simulink model "Powertrain_Comparison"  (R2024b)
settings: Solver=FixedStepDiscrete  StartTime=0.0  StopTime=3600  FixedStep=1  RelTol=1e-3
InitFcn:
  | try; sc=find_system(bdroot,'LookUnderMasks','all','FollowLinks','on','BlockType','Scope'); for k=1:numel(sc); c=get_param(sc{k},'ScopeConfiguration'); try; c.AxesScaling='Auto'; catch; end; try; nd=prod(c.LayoutDimensions); catch; nd=1; end; for d=1:nd; try; c.ActiveDisplay=d; catch; end; try; c.ShowLegend=true; catch; end; end; end; catch; end
(part 4 of 4)

== system Powertrain_Comparison/Electric powertrain/Battery storage/Battery management/Stored_energy_inventory ==
  note: Stored energy inventory
  note: OUTPUTS AND MONITORING
  SOC_fraction : Inport  PortDimensions=1
  OCV_segment_1 : Fcn  Expr=ocv_cell_V(1)*(((((u(1)-ocv_soc(1))+abs(u(1)-ocv_soc(1)))/2)+(ocv_soc(2)-ocv_soc(1))-abs((((u(1)-ocv_soc(1))+abs(u(1)-ocv_soc(1)))/2)-(ocv_soc(2)-ocv_soc(1))))/2)+0.5*(ocv_cell_V(2)-ocv_cell_V(1))/(ocv_soc(2)-ocv_soc(1))*(((((u(1)-ocv_soc(1))+abs(u(1)-ocv_soc(1)))/2)+(ocv_soc(2)-ocv_soc(1))-abs((((u(1)-ocv_soc(1))+abs(u(1)-ocv_soc(1)))/2)-(ocv_soc(2)-ocv_soc(1))))/2)^2
  OCV_segment_10 : Fcn  Expr=ocv_cell_V(10)*(((((u(1)-ocv_soc(10))+abs(u(1)-ocv_soc(10)))/2)+(ocv_soc(11)-ocv_soc(10))-abs((((u(1)-ocv_soc(10))+abs(u(1)-ocv_soc(10)))/2)-(ocv_soc(11)-ocv_soc(10))))/2)+0.5*(ocv_cell_V(11)-ocv_cell_V(10))/(ocv_soc(11)-ocv_soc(10))*(((((u(1)-ocv_soc(10))+abs(u(1)-ocv_soc(10)))/2)+(ocv_soc(11)-ocv_soc(10))-abs((((u(1)-ocv_soc(10))+abs(u(1)-ocv_soc(10)))/2)-(ocv_soc(11)-ocv_soc(10))))/2)^2
  OCV_segment_11 : Fcn  Expr=ocv_cell_V(11)*(((((u(1)-ocv_soc(11))+abs(u(1)-ocv_soc(11)))/2)+(ocv_soc(12)-ocv_soc(11))-abs((((u(1)-ocv_soc(11))+abs(u(1)-ocv_soc(11)))/2)-(ocv_soc(12)-ocv_soc(11))))/2)+0.5*(ocv_cell_V(12)-ocv_cell_V(11))/(ocv_soc(12)-ocv_soc(11))*(((((u(1)-ocv_soc(11))+abs(u(1)-ocv_soc(11)))/2)+(ocv_soc(12)-ocv_soc(11))-abs((((u(1)-ocv_soc(11))+abs(u(1)-ocv_soc(11)))/2)-(ocv_soc(12)-ocv_soc(11))))/2)^2
  OCV_segment_12 : Fcn  Expr=ocv_cell_V(12)*(((((u(1)-ocv_soc(12))+abs(u(1)-ocv_soc(12)))/2)+(ocv_soc(13)-ocv_soc(12))-abs((((u(1)-ocv_soc(12))+abs(u(1)-ocv_soc(12)))/2)-(ocv_soc(13)-ocv_soc(12))))/2)+0.5*(ocv_cell_V(13)-ocv_cell_V(12))/(ocv_soc(13)-ocv_soc(12))*(((((u(1)-ocv_soc(12))+abs(u(1)-ocv_soc(12)))/2)+(ocv_soc(13)-ocv_soc(12))-abs((((u(1)-ocv_soc(12))+abs(u(1)-ocv_soc(12)))/2)-(ocv_soc(13)-ocv_soc(12))))/2)^2
  OCV_segment_2 : Fcn  Expr=ocv_cell_V(2)*(((((u(1)-ocv_soc(2))+abs(u(1)-ocv_soc(2)))/2)+(ocv_soc(3)-ocv_soc(2))-abs((((u(1)-ocv_soc(2))+abs(u(1)-ocv_soc(2)))/2)-(ocv_soc(3)-ocv_soc(2))))/2)+0.5*(ocv_cell_V(3)-ocv_cell_V(2))/(ocv_soc(3)-ocv_soc(2))*(((((u(1)-ocv_soc(2))+abs(u(1)-ocv_soc(2)))/2)+(ocv_soc(3)-ocv_soc(2))-abs((((u(1)-ocv_soc(2))+abs(u(1)-ocv_soc(2)))/2)-(ocv_soc(3)-ocv_soc(2))))/2)^2
  OCV_segment_3 : Fcn  Expr=ocv_cell_V(3)*(((((u(1)-ocv_soc(3))+abs(u(1)-ocv_soc(3)))/2)+(ocv_soc(4)-ocv_soc(3))-abs((((u(1)-ocv_soc(3))+abs(u(1)-ocv_soc(3)))/2)-(ocv_soc(4)-ocv_soc(3))))/2)+0.5*(ocv_cell_V(4)-ocv_cell_V(3))/(ocv_soc(4)-ocv_soc(3))*(((((u(1)-ocv_soc(3))+abs(u(1)-ocv_soc(3)))/2)+(ocv_soc(4)-ocv_soc(3))-abs((((u(1)-ocv_soc(3))+abs(u(1)-ocv_soc(3)))/2)-(ocv_soc(4)-ocv_soc(3))))/2)^2
  OCV_segment_4 : Fcn  Expr=ocv_cell_V(4)*(((((u(1)-ocv_soc(4))+abs(u(1)-ocv_soc(4)))/2)+(ocv_soc(5)-ocv_soc(4))-abs((((u(1)-ocv_soc(4))+abs(u(1)-ocv_soc(4)))/2)-(ocv_soc(5)-ocv_soc(4))))/2)+0.5*(ocv_cell_V(5)-ocv_cell_V(4))/(ocv_soc(5)-ocv_soc(4))*(((((u(1)-ocv_soc(4))+abs(u(1)-ocv_soc(4)))/2)+(ocv_soc(5)-ocv_soc(4))-abs((((u(1)-ocv_soc(4))+abs(u(1)-ocv_soc(4)))/2)-(ocv_soc(5)-ocv_soc(4))))/2)^2
  OCV_segment_5 : Fcn  Expr=ocv_cell_V(5)*(((((u(1)-ocv_soc(5))+abs(u(1)-ocv_soc(5)))/2)+(ocv_soc(6)-ocv_soc(5))-abs((((u(1)-ocv_soc(5))+abs(u(1)-ocv_soc(5)))/2)-(ocv_soc(6)-ocv_soc(5))))/2)+0.5*(ocv_cell_V(6)-ocv_cell_V(5))/(ocv_soc(6)-ocv_soc(5))*(((((u(1)-ocv_soc(5))+abs(u(1)-ocv_soc(5)))/2)+(ocv_soc(6)-ocv_soc(5))-abs((((u(1)-ocv_soc(5))+abs(u(1)-ocv_soc(5)))/2)-(ocv_soc(6)-ocv_soc(5))))/2)^2
  OCV_segment_6 : Fcn  Expr=ocv_cell_V(6)*(((((u(1)-ocv_soc(6))+abs(u(1)-ocv_soc(6)))/2)+(ocv_soc(7)-ocv_soc(6))-abs((((u(1)-ocv_soc(6))+abs(u(1)-ocv_soc(6)))/2)-(ocv_soc(7)-ocv_soc(6))))/2)+0.5*(ocv_cell_V(7)-ocv_cell_V(6))/(ocv_soc(7)-ocv_soc(6))*(((((u(1)-ocv_soc(6))+abs(u(1)-ocv_soc(6)))/2)+(ocv_soc(7)-ocv_soc(6))-abs((((u(1)-ocv_soc(6))+abs(u(1)-ocv_soc(6)))/2)-(ocv_soc(7)-ocv_soc(6))))/2)^2
  OCV_segment_7 : Fcn  Expr=ocv_cell_V(7)*(((((u(1)-ocv_soc(7))+abs(u(1)-ocv_soc(7)))/2)+(ocv_soc(8)-ocv_soc(7))-abs((((u(1)-ocv_soc(7))+abs(u(1)-ocv_soc(7)))/2)-(ocv_soc(8)-ocv_soc(7))))/2)+0.5*(ocv_cell_V(8)-ocv_cell_V(7))/(ocv_soc(8)-ocv_soc(7))*(((((u(1)-ocv_soc(7))+abs(u(1)-ocv_soc(7)))/2)+(ocv_soc(8)-ocv_soc(7))-abs((((u(1)-ocv_soc(7))+abs(u(1)-ocv_soc(7)))/2)-(ocv_soc(8)-ocv_soc(7))))/2)^2
  OCV_segment_8 : Fcn  Expr=ocv_cell_V(8)*(((((u(1)-ocv_soc(8))+abs(u(1)-ocv_soc(8)))/2)+(ocv_soc(9)-ocv_soc(8))-abs((((u(1)-ocv_soc(8))+abs(u(1)-ocv_soc(8)))/2)-(ocv_soc(9)-ocv_soc(8))))/2)+0.5*(ocv_cell_V(9)-ocv_cell_V(8))/(ocv_soc(9)-ocv_soc(8))*(((((u(1)-ocv_soc(8))+abs(u(1)-ocv_soc(8)))/2)+(ocv_soc(9)-ocv_soc(8))-abs((((u(1)-ocv_soc(8))+abs(u(1)-ocv_soc(8)))/2)-(ocv_soc(9)-ocv_soc(8))))/2)^2
  OCV_segment_9 : Fcn  Expr=ocv_cell_V(9)*(((((u(1)-ocv_soc(9))+abs(u(1)-ocv_soc(9)))/2)+(ocv_soc(10)-ocv_soc(9))-abs((((u(1)-ocv_soc(9))+abs(u(1)-ocv_soc(9)))/2)-(ocv_soc(10)-ocv_soc(9))))/2)+0.5*(ocv_cell_V(10)-ocv_cell_V(9))/(ocv_soc(10)-ocv_soc(9))*(((((u(1)-ocv_soc(9))+abs(u(1)-ocv_soc(9)))/2)+(ocv_soc(10)-ocv_soc(9))-abs((((u(1)-ocv_soc(9))+abs(u(1)-ocv_soc(9)))/2)-(ocv_soc(10)-ocv_soc(9))))/2)^2
  Pack_stored_energy_kWh : Gain  Gain=ns*np*cell_capacity_Ah/1000  SaturateOnIntegerOverflow=on  OutDataTypeStr=Inherit: Same as input  ParamDataTypeStr=Inherit: Same as input
  Sum_segment_voltage_integrals : Sum  Inputs=++++++++++++  InputSameDT=on  SaturateOnIntegerOverflow=on  OutDataTypeStr=Inherit: Same as first input
  Stored_energy_kWh : Outport
  wires:
  OCV_segment_5/1 -> Sum_segment_voltage_integrals/5
  SOC_fraction/1 -> OCV_segment_1/1, OCV_segment_2/1, OCV_segment_3/1, OCV_segment_4/1, OCV_segment_8/1, OCV_segment_6/1, OCV_segment_9/1, OCV_segment_10/1, OCV_segment_5/1, OCV_segment_11/1, OCV_segment_12/1, OCV_segment_7/1
  OCV_segment_6/1 -> Sum_segment_voltage_integrals/6
  OCV_segment_2/1 -> Sum_segment_voltage_integrals/2
  OCV_segment_1/1 -> Sum_segment_voltage_integrals/1
  OCV_segment_7/1 -> Sum_segment_voltage_integrals/7
  OCV_segment_3/1 -> Sum_segment_voltage_integrals/3
  OCV_segment_4/1 -> Sum_segment_voltage_integrals/4
  OCV_segment_8/1 -> Sum_segment_voltage_integrals/8
  OCV_segment_9/1 -> Sum_segment_voltage_integrals/9
  OCV_segment_10/1 -> Sum_segment_voltage_integrals/10
  OCV_segment_11/1 -> Sum_segment_voltage_integrals/11
  OCV_segment_12/1 -> Sum_segment_voltage_integrals/12
  Sum_segment_voltage_integrals/1 -> Pack_stored_energy_kWh/1
  Pack_stored_energy_kWh/1 -> Stored_energy_kWh/1
